simulink model "step2_cell"  (R2025b)
settings: Solver=VariableStepAuto  StartTime=0.0  StopTime=t_end  MaxStep=1  RelTol=1e-3
InitFcn:
  | step2_params;
values from neighbouring files (symbols this model uses):
  I_pulse = 4    [step2_params.m]
  ocv_table = [3.00 3.45 3.55 3.62 3.68 3.75 3.85 3.95 4.05 4.12 4.20]    [step1_single_cell.m]    (also in step2_params.m)
  Q = Q_Ah * 3600    (= 9000)    [step1_single_cell.m]    (also in step2_params.m)
  R0 = 0.030    (= 0.03)    [step1_single_cell.m]    (also in step2_params.m)
  SOC0 = 1.0    (= 1)    [step2_params.m]
  soc_table = 0:0.1:1    [step1_single_cell.m]    (also in step2_params.m)
  T_cycle = 600    [step2_params.m]
settings Model: Creator=Saquire  LastModifiedBy=Saquire

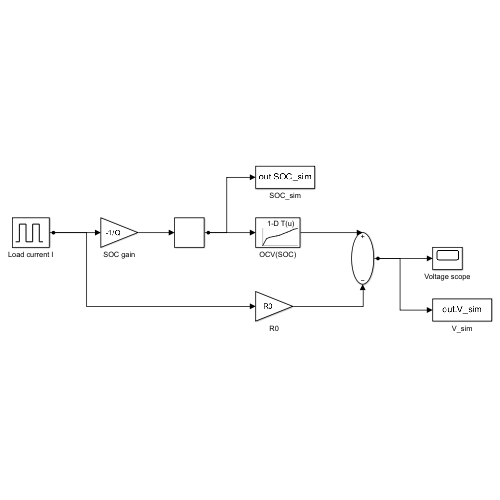
[thumbnail: Simulink's stored preview of the top-level diagram]
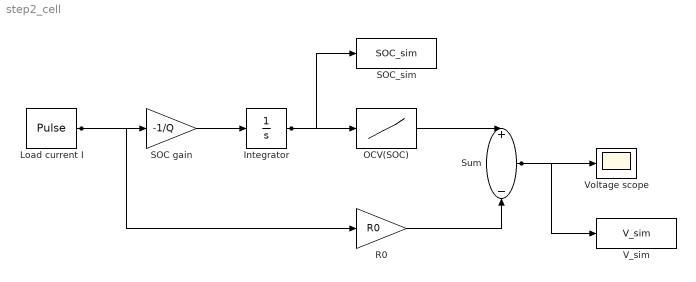
== system step2_cell ==
  Integrator : Integrator  InitialCondition=SOC0
  Load current I : DiscretePulseGenerator  PulseType=Time based  Amplitude=I_pulse  Period=T_cycle  PulseWidth=50
  OCV(SOC) : Lookup_n-D  NumberOfTableDimensions=1  BreakpointsForDimension1=soc_table  Table=ocv_table  InternalRulePriority=Speed  RndMeth=Simplest
  R0 : Gain  Gain=R0
  SOC gain : Gain  Gain=-1/Q
  SOC_sim : ToWorkspace  VariableName=SOC_sim  SaveFormat=Timeseries  SampleTime=-1
  Sum : Sum  Inputs=+-
  V_sim : ToWorkspace  VariableName=V_sim  SaveFormat=Timeseries  SampleTime=-1
  Voltage scope : Scope
  wires:
  Load current I/1 -> SOC gain/1, R0/1
  SOC gain/1 -> Integrator/1
  Integrator/1 -> OCV(SOC)/1, SOC_sim/1
  OCV(SOC)/1 -> Sum/1
  R0/1 -> Sum/2
  Sum/1 -> Voltage scope/1, V_sim/1
